simulink model "walec_ostroslup_simulink"  (R2025b)
settings: Solver=VariableStepAuto  StartTime=0.0  StopTime=10.0  RelTol=1e-3
values from neighbouring files (symbols this model uses):
  A2 = 1.47044    [walec_ostroslup.m]
  B2 = 4.08042    [walec_ostroslup.m]
  C1 = 1.8257    [walec_ostroslup.m]
  C2 = 0.745356    [walec_ostroslup.m]
  H2 = 10    [walec_ostroslup.m]
  R1 = 1.9544    [walec_ostroslup.m]
settings Model: Creator=Matadoo  LastModifiedBy=wystr

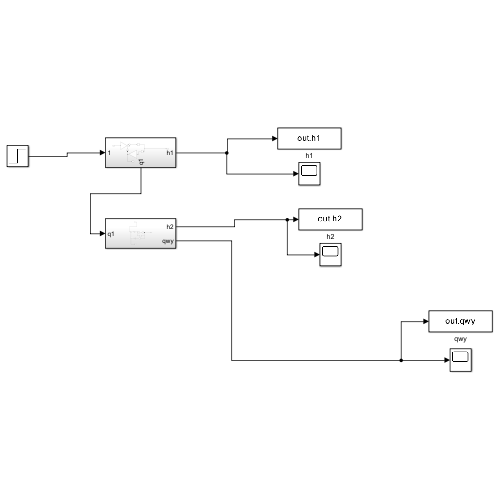
[thumbnail: Simulink's stored preview of the top-level diagram]
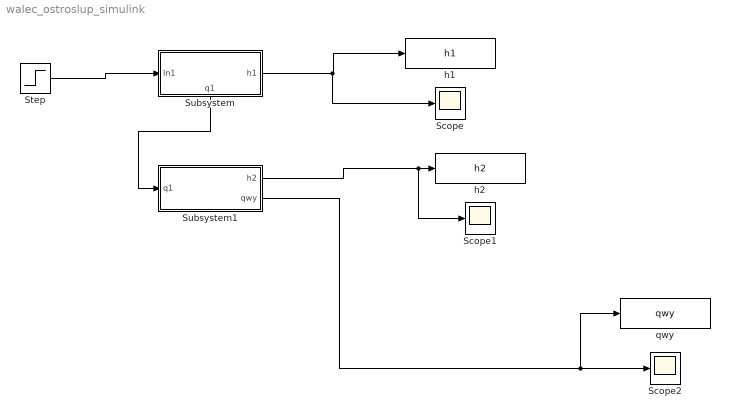
== system walec_ostroslup_simulink ==
  Scope : Scope
      settings: ActiveDisplayYMinimum=-1  ActiveDisplayYMaximum=1
  Scope1 : Scope
      settings: ActiveDisplayYMinimum=0.54521  ActiveDisplayYMaximum=9.07763
  Scope2 : Scope
      settings: ActiveDisplayYMinimum=0.53358  ActiveDisplayYMaximum=1.45875  DataLoggingVariableName=ScopeData2
  Step : Step  SampleTime=0
  Subsystem : Subsystem
      settings: PortSchema="{\"entries\":[{\"content\":{\"sides\":[{\"content\":{\"connectorIds\":[\"In1\"]},\"type\":\"ConnectorPlacement.EquallySpacedRectSide\",\"uuid\":\"ef9d34a5-cff8-451d-8a8e-ad43d62a4229\"},{\"content\":{\"connectorIds\":[\"Out1\"],\"side\":\"RIGHT\"},\"type\":\"ConnectorPlacement.EquallySpacedRectSide\",\"uuid\":\"a0647498-08a7-49d7-b729-cb433a3947bd\"},{\"content\":{\"side\":\"TOP\"},\"type\":\"ConnectorPlacement.EquallySpacedRectSide\",\"uuid\":\"e54223c9-a9e4-45b8-9f51-507c5557501a\"},{\"content\":{\"connectorIds\":[\"Out2\"],\"side\":\"BOTTOM\"},\"type\":\"ConnectorPlacement.EquallySpacedRectSide\",\"uuid\":\"7d5bf5b3-bf67-4990-a720-c5a5b654a001\"}]},\"type\":\"ConnectorPlacement.EquallySpacedConnector\",\"uuid\":\"879e1674-e5d1-4532-ab14-c8e474c4df17\"}],\"packageUris\":[\"http://schema.mathworks.com/mf0/Connector/R2020b\"],\"version\":\"1.0\"}"
  Subsystem1 : Subsystem
  h1 : ToWorkspace  VariableName=h1  SampleTime=-1
      settings: Save2DSignal=2-D array (concatenate along first dimension)
  h2 : ToWorkspace  VariableName=h2  SampleTime=-1
      settings: Save2DSignal=2-D array (concatenate along first dimension)
  qwy : ToWorkspace  VariableName=qwy  SampleTime=-1
      settings: Save2DSignal=2-D array (concatenate along first dimension)
  wires:
  Subsystem/2(q1) -> Subsystem1/1(q1)
  Subsystem/1(h1) -> Scope/1, h1/1
  Subsystem1/1(h2) -> Scope1/1, h2/1
  Subsystem1/2(qwy) -> qwy/1, Scope2/1
  Step/1 -> Subsystem/1(In1)

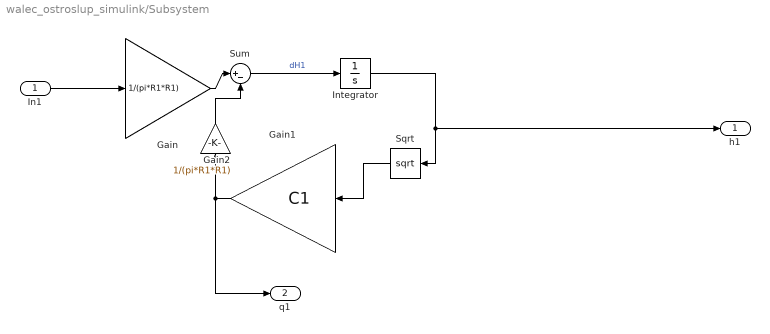
== system walec_ostroslup_simulink/Subsystem ==
  In1 : Inport
  Gain : Gain  Gain=1/(pi*R1*R1)
  Gain1 : Gain  Gain=C1
  Gain2 : Gain  Gain=1/(pi*R1*R1)
  Integrator : Integrator
  Sqrt : Sqrt
  Sum : Sum  Inputs=|+-
  h1 : Outport
  q1 : Outport  Port=2
  wires:
  Gain/1 -> Sum/1
  Integrator/1 -> h1/1, Sqrt/1
  Sqrt/1 -> Gain1/1
  Gain1/1 -> Gain2/1, q1/1
  Sum/1 -> Integrator/1  "dH1"
  In1/1 -> Gain/1
  Gain2/1 -> Sum/2

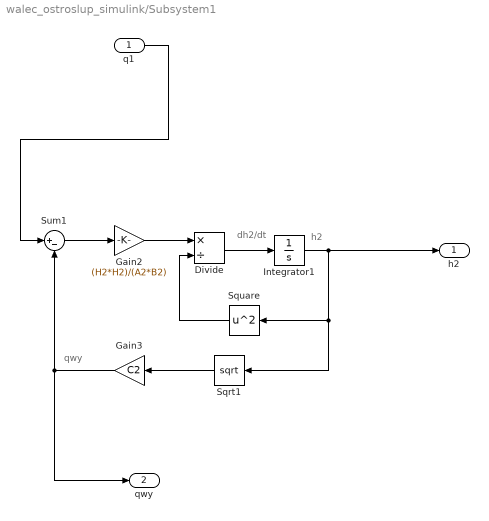
== system walec_ostroslup_simulink/Subsystem1 ==
  note: qwy
  note: dh2/dt
  note: h2
  q1 : Inport
  Divide : Product  Inputs=*/
  Gain2 : Gain  Gain=(H2*H2)/(A2*B2)
  Gain3 : Gain  Gain=C2
  Integrator1 : Integrator  InitialCondition=0.1*H2
  Sqrt1 : Sqrt
  Square : Math  Operator=square
  Sum1 : Sum  Inputs=|+-
  h2 : Outport
  qwy : Outport  Port=2
  wires:
  Sum1/1 -> Gain2/1
  Gain3/1 -> qwy/1, Sum1/2
  Square/1 -> Divide/2
  Divide/1 -> Integrator1/1
  Gain2/1 -> Divide/1
  Integrator1/1 -> h2/1, Sqrt1/1, Square/1
  q1/1 -> Sum1/1
  Sqrt1/1 -> Gain3/1
